simulink model "eksperiment_pid_regulacija"  (R2015b)
settings: Solver=VariableStepAuto  StartTime=0.0  StopTime=inf  RelTol=1e-3
undefined symbols (not defined in the file): analoginput, analogoutput
libraries: daqlib x2, simulink x1
settings Model: Creator=admin  LastModifiedBy=Elma

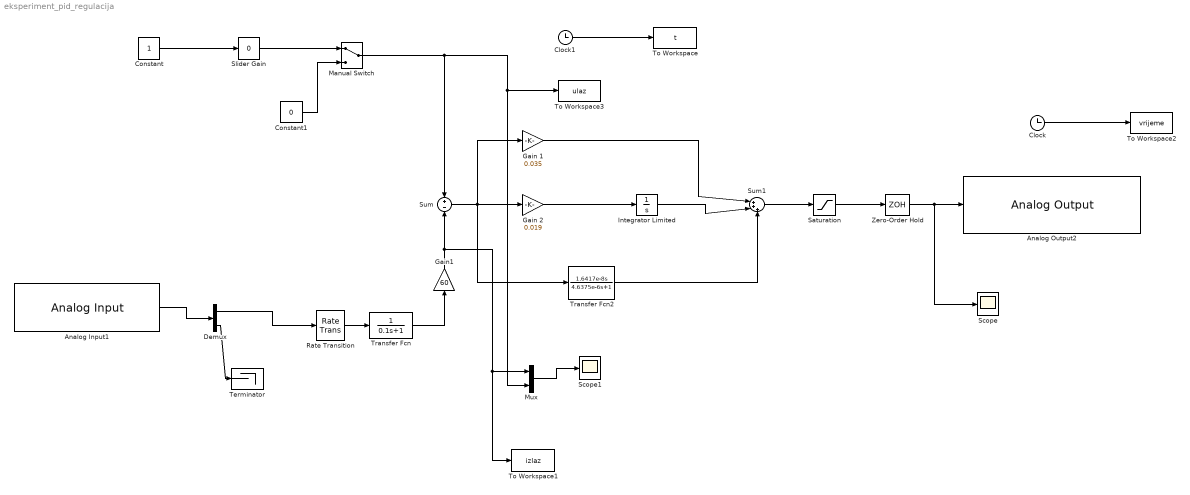
== system eksperiment_pid_regulacija ==
  Analog Input1 : daqlib/Analog Input  AcqMode=0  DeviceMenu=winsound 0 (Microphone Array (Intel?)  Device=nidaq Dev1 (PCI-6024E)  ObjConstructor=analoginput('nidaq','Dev1')  SampleRate=1000  ActualRate=1000  SamplesPerFrame=2  InputType=SingleEnded  NChannelsSelected=1  Channels=0$0$$1$#0$1$$1$#0$2$$1$#0$3$$1$#0$4$$1$#0$5$$1$#1$6$$1$#0$7$$1$#0$8$$1$#0$9$$1$#0$10$$1$#0$11$$1$#0$12$$1$#0$13$$1$#0$14$$1$#0$15$$1$#  NPorts=1 per hardware channel  DataType=double
      settings: SignalType=Sample-based
  Analog Output2 : daqlib/Analog Output  OutMode=0  DeviceMenu=winsound 0 (Microphone Array (Intel?)  Device=nidaq Dev1 (PCI-6024E)  ObjConstructor=analogoutput('nidaq','Dev1')  OutputRate=1000  ActualRate=1000  NChannelsSelected=1  Channels=1$0$$1$0$#0$1$$1$0$#  NPorts=1 per hardware channel
  Clock : Clock
  Clock1 : Clock
  Constant : Constant
  Constant1 : Constant  Value=0
  Demux : Demux  Outputs=2
  Gain 1 : Gain  Gain=0.035
  Gain 2 : Gain  Gain=0.019
  Gain1 : Gain  Gain=60
  Integrator Limited : Integrator  LimitOutput=on  UpperSaturationLimit=10  LowerSaturationLimit=0
  Manual Switch : ManualSwitch
  Mux : Mux  Inputs=2
  Rate Transition : RateTransition
  Saturation : Saturate  UpperLimit=10  LowerLimit=0
  Scope : Scope
  Scope1 : Scope
  Slider Gain : simulink/Math Operations/Slider Gain  low=0  gain=0  high=60
  Sum : Sum  Inputs=+-
  Sum1 : Sum  Inputs=|+++
  Terminator : Terminator
  To Workspace : ToWorkspace  VariableName=t  SampleTime=-1
      settings: Save2DSignal=2-D array (concatenate along first dimension)
  To Workspace1 : ToWorkspace  VariableName=izlaz  SampleTime=-1
      settings: Save2DSignal=2-D array (concatenate along first dimension)
  To Workspace2 : ToWorkspace  VariableName=vrijeme  SampleTime=-1
      settings: Save2DSignal=2-D array (concatenate along first dimension)
  To Workspace3 : ToWorkspace  VariableName=ulaz  SampleTime=-1
      settings: Save2DSignal=2-D array (concatenate along first dimension)
  Transfer Fcn : TransferFcn  Denominator=[0.1 1]
  Transfer Fcn2 : TransferFcn  Numerator=[1.6417e-8 0]  Denominator=[4.6375e-6 1]
  Zero-Order Hold : ZeroOrderHold  SampleTime=0.001
  wires:
  Sum/1 -> Transfer Fcn2/1, Gain 1/1, Gain 2/1
  Gain 1/1 -> Sum1/1
  Integrator Limited/1 -> Sum1/2
  Sum1/1 -> Saturation/1
  Gain 2/1 -> Integrator Limited/1
  Clock/1 -> To Workspace2/1
  Constant/1 -> Slider Gain/1
  Analog Input1/1 -> Demux/1
  Demux/1 -> Rate Transition/1
  Demux/2 -> Terminator/1
  Rate Transition/1 -> Transfer Fcn/1
  Saturation/1 -> Zero-Order Hold/1
  Zero-Order Hold/1 -> Analog Output2/1, Scope/1
  Slider Gain/1 -> Manual Switch/1
  Constant1/1 -> Manual Switch/2
  Manual Switch/1 -> Mux/2, To Workspace3/1, Sum/1
  Transfer Fcn/1 -> Gain1/1
  Gain1/1 -> To Workspace1/1, Mux/1, Sum/2
  Mux/1 -> Scope1/1
  Transfer Fcn2/1 -> Sum1/3
  Clock1/1 -> To Workspace/1
